simulink model "svpwm_inv_ideal_switch_drive"  (R2025a)
settings: Solver=daessc  StartTime=0.0  StopTime=1  MaxStep=2.5e-7  RelTol=1e-3
model workspace (MAT data in the model file):
  FocDiscrTime = 0.0001
  Is_max = 450
  Ld = 0.00031
  Lq = 0.000305
  PolePairs = 11
  Psi = 0.09569
  Rs = 0.02
  VDC = 400
  compensate_dt = 0
  compensate_pwm = 0
  piBandwidth = 5000
undefined symbols (not defined in the file): Down, Up
libraries: fl_lib x20, nesl_utility x19, ee_lib x15, mcbeeMathTransformLib x7, spsMeanLib x7, slpidlib x5, eePwmGenerator x3, spsRMSLib x2, simulink x2, simulink_extras x1
(part 1 of 2)
settings Model: SimulationMode=rapid-accelerator  ExtModeTrigDuration=100  ParameterArgumentNames=FocDiscrTime  Creator=alexey  LastModifiedBy=alexey
settings SolverCC: ZeroCrossAlgorithm=Adaptive
settings OptimizationCC: DefaultParameterBehavior=Inlined  UseDivisionForNetSlopeComputation=on  GainParamInheritBuiltInType=on  UseFloatMulNetSlope=on  InlineInvariantSignals=on  ReuseModelBlockBuffer=off  EfficientFloat2IntCast=on  LifeSpan=1
settings DebuggingCC: IgnoredZcDiagnostic=none
settings HardwareCC: ProdLongLongMode=on
settings SFSimCC: MATLABDynamicMemAlloc=off
settings RTWCC: GenerateReport=on  LaunchReport=on  GPUComputeCapability=3.5
settings CodeAppCC: ForceParamTrailComments=on
settings GRTTargetCC: RTWCAPISignals=on  RTWCAPIParams=on  CombineSignalStateStructs=on  MatFileLogging=off  SupportVariableSizeSignals=on

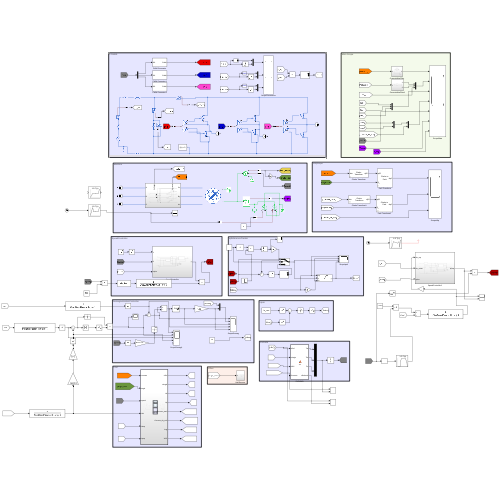
[thumbnail: Simulink's stored preview of the top-level diagram]
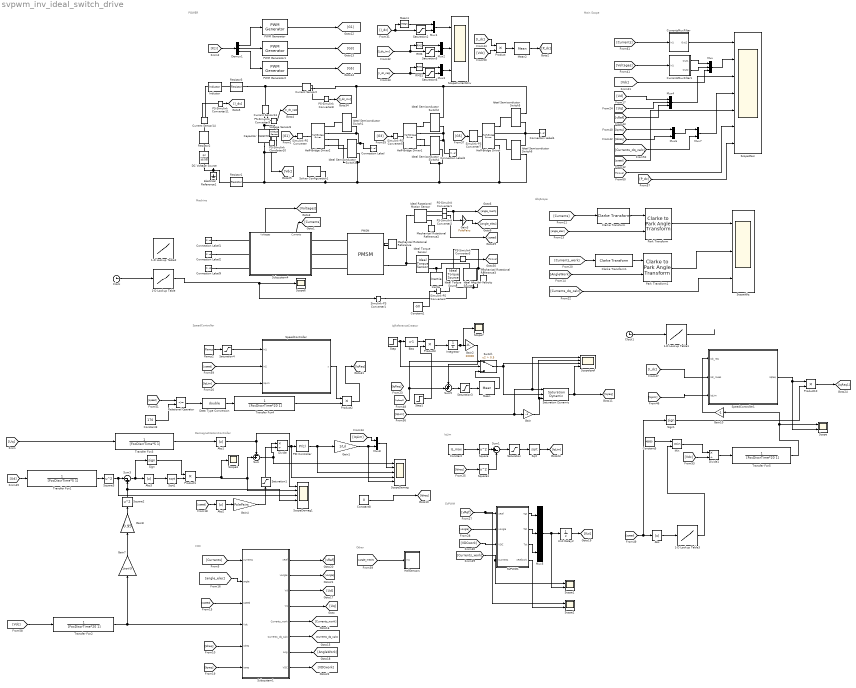
== system svpwm_inv_ideal_switch_drive ==
  note: POWER
  note: IqLim
  note: DemagnetizationController
  note: FOC
  note: Machine
  note: SpeedController
  note: Other
  note: Main Scope
  note: IqReferenceCreator
  note: IdIqScope
  note: SVPWM
  1-D Lookup Table : Lookup_n-D  NumberOfTableDimensions=1  BreakpointsForDimension1=[0 0.4 0.45 0.55 0.87 1 1.5 1.6 1.7]  Table=[0 208 208 104 104 120 120 220 220]  InternalRulePriority=Speed  RndMeth=Simplest
  1-D Lookup Table1 : Lookup_n-D  NumberOfTableDimensions=1  BreakpointsForDimension1=[0 0.3 1 1.2 1.3 1.4 1.5]  Table=[0 200 150 200 30 250 250]  InternalRulePriority=Speed  RndMeth=Simplest
  1-D Lookup Table2 : Lookup_n-D  NumberOfTableDimensions=1  BreakpointsForDimension1=[0 0.4 0.45 0.55 0.87 1 1.5 1.6 1.7]  Table=[0 104 104 104 104 120 120 220 220]  InternalRulePriority=Speed  RndMeth=Simplest
  1-D Lookup Table3 : Lookup_n-D  NumberOfTableDimensions=1  BreakpointsForDimension1=[0 550 600 1000 1925 2350 2400 2450]*0.1047  Table=[0 0 30000 48500 48500 22000 0 0]  InternalRulePriority=Speed  RndMeth=Simplest
  Abs{,1..3} (4 alike) : Abs  SaturateOnIntegerOverflow=off
  Bias : Bias  Bias=-1  SaturateOnIntegerOverflow=off
  Capacitor : fl_lib/Electrical/Electrical Elements/Capacitor  c=300 uF  r=1 mOhm  g=0 1/Ohm  i_specify=off  i_priority=None  i=0 A  i_nominal_specify=off  i_nominal_value=1  i_nominal_unit=A  v_specify=off  v_priority=High  v=400 V  v_nominal_specify=off  v_nominal_value=1  v_nominal_unit=V  vc_specify=on  vc_priority=High  vc=VDC V  vc_nominal_specify=off  vc_nominal_value=1  vc_nominal_unit=V
  Clarke Transform : mcbeeMathTransformLib/Clarke Transform  VariantControl=Variant2  PowerInvariant=off  UseWithEmbedded=on  PhaseInput=Three inputs
      settings: LibrarySourceBlock=mcbcontrolslib/Clarke Transform
  Clarke Transform1 : mcbeeMathTransformLib/Clarke Transform  VariantControl=Variant2  PowerInvariant=off  UseWithEmbedded=on  PhaseInput=Three inputs
      settings: LibrarySourceBlock=mcbcontrolslib/Clarke Transform
  Clock : Clock
  Clock1 : Clock
  Connection Label : ConnectionLabel  Label=A
  Connection Label1 : ConnectionLabel  Label=A
  Connection Label2 : ConnectionLabel  Label=B
  Connection Label3 : ConnectionLabel  Label=B
  Connection Label4 : ConnectionLabel  Label=C
  Connection Label9 : ConnectionLabel  Label=C
  Constant : Constant  Value=Is_max
  Constant1 : Constant  Value=-50
  Constant3 : Constant  Value=170
  Constant5 : Constant  Value=48500
  Constant8 : Constant  Value=0
  Current Sensor13 : fl_lib/Electrical/Electrical Sensors/Current Sensor
  Current Sensor14 : fl_lib/Electrical/Electrical Sensors/Current Sensor
  Current Sensor2 : fl_lib/Electrical/Electrical Sensors/Current Sensor
  CurrentsMuxFilter : Subsystem
  CurrentsMuxFilter1 : Subsystem
  DC Voltage Source : ee_lib/Additional Components/SPICE Sources/DC Voltage Source  DC=VDC V
  Data Type Conversion : DataTypeConversion  OutDataTypeStr=double  SaturateOnIntegerOverflow=off  RndMeth=Floor
  Demux1 : Demux  Outputs=3
  Divide : Product  Inputs=*/
  Divide1 : Product  Inputs=*/
  Electrical Reference1 : fl_lib/Electrical/Electrical Elements/Electrical Reference
  Gain : Gain  Gain=-1
  Gain1 : Gain  Gain=1/Ld
  Gain10 : Gain  Gain=-1
  Gain2 : Gain  Gain=20000
  Gain3 : Gain  Gain=PolePairs
  Gain4 : Gain  Gain=PolePairs
  Gain7 : Gain  Gain=1/sqrt(3)
  Gain8 : Gain  Gain=0.95
  Half-Bridge Driver : ee_lib/Semiconductors & Converters/Half-Bridge Driver  port_option=ee.enum.controlport.ps  uHigh=2.0 V  uLow=0.8 V  uHighValue=0.7  uLowValue=0.3  vHigh=15 V  vLow=0 V  tpLH=50 ns  tdLH=1 ns  tpHL=50 ns  tdHL=1 ns  parameterization=ee.enum.semiconductors.gateDriverParam.outputImpedance  rHigh=2 Ohm  rLow=2 Ohm  tRise=20 ns  tFall=20 ns  cLoad=10 nF  ZonTime_specify=off  ZonTime_priority=None  ZonTime=0 s  ZoffTime_specify=off  ZoffTime_priority=None  ZoffTime=0 s  power_dissipated_high_side_specify=off  power_dissipated_high_side_priority=None  power_dissipated_high_side=0 W  power_dissipated_high_side_nominal_specify=off  power_dissipated_high_side_nominal_value=1  power_dissipated_high_side_nominal_unit=W  power_dissipated_low_side_specify=off  power_dissipated_low_side_priority=None  power_dissipated_low_side=0 W  power_dissipated_low_side_nominal_specify=off  power_dissipated_low_side_nominal_value=1  power_dissipated_low_side_nominal_unit=W
      settings: InternalSimscapePortConfiguration="{\"Bottom\":[],\"Left\":[{\"id\":\"u\",\"label\":\"u\",\"type\":\"input\"}],\"Right\":[{\"id\":\"HO\",\"label\":\"HO\",\"type\":\"foundation.electrical.electrical\"},{\"id\":\"HS\",\"label\":\"HS\",\"type\":\"foundation.electrical.electrical\"},{\"id\":\"LO\",\"label\":\"LO\",\"type\":\"foundation.electrical.electrical\"},{\"id\":\"LS\",\"label\":\"LS\",\"type\":\"foundation.electrical.electrical\"}],\"Top\":[]}"
  Half-Bridge Driver1 : ee_lib/Semiconductors & Converters/Half-Bridge Driver  port_option=ee.enum.controlport.ps  uHigh=2.0 V  uLow=0.8 V  uHighValue=0.7  uLowValue=0.3  vHigh=15 V  vLow=0 V  tpLH=50 ns  tdLH=1 ns  tpHL=50 ns  tdHL=1 ns  parameterization=ee.enum.semiconductors.gateDriverParam.outputImpedance  rHigh=2 Ohm  rLow=2 Ohm  tRise=20 ns  tFall=20 ns  cLoad=10 nF  ZonTime_specify=off  ZonTime_priority=None  ZonTime=0 s  ZoffTime_specify=off  ZoffTime_priority=None  ZoffTime=0 s  power_dissipated_high_side_specify=off  power_dissipated_high_side_priority=None  power_dissipated_high_side=0 W  power_dissipated_high_side_nominal_specify=off  power_dissipated_high_side_nominal_value=1  power_dissipated_high_side_nominal_unit=W  power_dissipated_low_side_specify=off  power_dissipated_low_side_priority=None  power_dissipated_low_side=0 W  power_dissipated_low_side_nominal_specify=off  power_dissipated_low_side_nominal_value=1  power_dissipated_low_side_nominal_unit=W
      settings: InternalSimscapePortConfiguration="{\"Bottom\":[],\"Left\":[{\"id\":\"u\",\"label\":\"u\",\"type\":\"input\"}],\"Right\":[{\"id\":\"HO\",\"label\":\"HO\",\"type\":\"foundation.electrical.electrical\"},{\"id\":\"HS\",\"label\":\"HS\",\"type\":\"foundation.electrical.electrical\"},{\"id\":\"LO\",\"label\":\"LO\",\"type\":\"foundation.electrical.electrical\"},{\"id\":\"LS\",\"label\":\"LS\",\"type\":\"foundation.electrical.electrical\"}],\"Top\":[]}"
  Half-Bridge Driver2 : ee_lib/Semiconductors & Converters/Half-Bridge Driver  port_option=ee.enum.controlport.ps  uHigh=2.0 V  uLow=0.8 V  uHighValue=0.7  uLowValue=0.3  vHigh=15 V  vLow=0 V  tpLH=50 ns  tdLH=1 ns  tpHL=50 ns  tdHL=1 ns  parameterization=ee.enum.semiconductors.gateDriverParam.outputImpedance  rHigh=2 Ohm  rLow=2 Ohm  tRise=20 ns  tFall=20 ns  cLoad=10 nF  ZonTime_specify=off  ZonTime_priority=None  ZonTime=0 s  ZoffTime_specify=off  ZoffTime_priority=None  ZoffTime=0 s  power_dissipated_high_side_specify=off  power_dissipated_high_side_priority=None  power_dissipated_high_side=0 W  power_dissipated_high_side_nominal_specify=off  power_dissipated_high_side_nominal_value=1  power_dissipated_high_side_nominal_unit=W  power_dissipated_low_side_specify=off  power_dissipated_low_side_priority=None  power_dissipated_low_side=0 W  power_dissipated_low_side_nominal_specify=off  power_dissipated_low_side_nominal_value=1  power_dissipated_low_side_nominal_unit=W
      settings: InternalSimscapePortConfiguration="{\"Bottom\":[],\"Left\":[{\"id\":\"u\",\"label\":\"u\",\"type\":\"input\"}],\"Right\":[{\"id\":\"HO\",\"label\":\"HO\",\"type\":\"foundation.electrical.electrical\"},{\"id\":\"HS\",\"label\":\"HS\",\"type\":\"foundation.electrical.electrical\"},{\"id\":\"LO\",\"label\":\"LO\",\"type\":\"foundation.electrical.electrical\"},{\"id\":\"LS\",\"label\":\"LS\",\"type\":\"foundation.electrical.electrical\"}],\"Top\":[]}"
  HallSensors : Subsystem
  Ideal Angular Velocity Source : fl_lib/Mechanical/Mechanical Sources/Ideal Angular Velocity Source
  Ideal Rotational Motion Sensor : fl_lib/Mechanical/Mechanical Sensors/Ideal Rotational Motion Sensor  reference=foundation.enum.MeasurementReference.difference  acceleration_port=false  velocity_port=true  position_port=true  wrap_angle=false  offset=0 rad
  Ideal Semiconductor Switch{1..6} (6 alike) : ee_lib/Semiconductors & Converters/Ideal Semiconductor Switch  port_option=ee.enum.controlport.elec  Ron=0.0001 Ohm  Goff=1e-6 1/Ohm  Vth=10 V  diode_param=ee.enum.semiconductors.protectionDiode.nodynamics  diode_Vf=0.8 V  diode_Ron=0.001 Ohm  diode_Goff=1e-5 1/Ohm  diode_C=50e-9 F  diode_iRM=-235 A  diode_iF=300 A  diode_idot=-50 A/us  diode_trr_param=ee.enum.converters.diodetrr.trr_factor  diode_trr_factor=3  diode_trr=15 us  diode_Qrr=1500 s*uA
      settings: InternalSimscapePortConfiguration="{\"Bottom\":[],\"Left\":[{\"id\":\"G_elec\",\"label\":\"\",\"type\":\"foundation.electrical.electrical\"}],\"Right\":[{\"id\":\"A\",\"label\":\"a\",\"type\":\"foundation.electrical.electrical\"},{\"id\":\"K\",\"label\":\"k\",\"type\":\"foundation.electrical.electrical\"}],\"Top\":[]}"
  Ideal Torque Sensor : fl_lib/Mechanical/Mechanical Sensors/Ideal Torque Sensor
  Ideal Torque Source : fl_lib/Mechanical/Mechanical Sources/Ideal Torque Source
  Inductor : ee_lib/Passive/Inductor  l=220e-9 H  enable_L_tol=ee.enum.toleranceApplication.none  L_tol=20  tol_distribution=ee.enum.toleranceDistribution.uniform  nSigma=4  r=0 Ohm  g=1e-9 1/Ohm  enable_operating_limits=ee.enum.enable.no  operating_limit_action=ee.enum.passive.reportOpLim.warn  max_working_current=1 A  power_rating=1 W  i_L_specify=off  i_L_priority=High  i_L=0 A  i_L_nominal_specify=off  i_L_nominal_value=1  i_L_nominal_unit=A
  Inertia : fl_lib/Mechanical/Rotational Elements/Inertia  inertia=0.1 kg*m^2  num_ports=foundation.enum.numPorts2.one  w_specify=off  w_priority=High  w=0 rad/s  w_nominal_specify=off  w_nominal_value=1  w_nominal_unit=rad/s  t_specify=off  t_priority=None  t=0 N*m  t_nominal_specify=off  t_nominal_value=1  t_nominal_unit=N*m
  Integrator : Integrator  LimitOutput=on  UpperSaturationLimit=0  LowerSaturationLimit=-2*Is_max/20000
  Mean : spsMeanLib/Mean  Freq=1000  Vinit=0  Ts=0
  Mean1 : spsMeanLib/Mean  Freq=1/FocDiscrTime/20  Vinit=0  Ts=0
  Mean2 : spsMeanLib/Mean  Freq=1/FocDiscrTime/20  Vinit=0  Ts=0
  Mechanical Rotational Reference : fl_lib/Mechanical/Rotational Elements/Mechanical Rotational Reference
  Mechanical Rotational Reference2 : fl_lib/Mechanical/Rotational Elements/Mechanical Rotational Reference
  Mechanical Rotational Reference3 : fl_lib/Mechanical/Rotational Elements/Mechanical Rotational Reference
  Min : MinMax  Inputs=2
  Mux : Mux  Inputs=3
  Mux{1..3,6..8} (6 alike) : Mux  Inputs=2
  Mux4 : Mux  Inputs=3
  Mux5 : Mux  Inputs=3
  PID Controller : slpidlib/PID Controller  Controller=PI  Form=Parallel  TimeDomain=Discrete-time  UseExternalTs=off  SampleTime=FocDiscrTime*10  IntegratorMethod=Forward Euler  FilterMethod=Forward Euler  ControllerParametersSource=internal  P=0.1*5  I=100*5  UseKiTs=off  D=0.01  UseExternalDerivativeSource=off  N=100  UseFilter=on  TunerSelectOption=Transfer Function Based (PID Tuner App)  InitialConditionSource=internal  InitialConditionForIntegrator=0  InitialConditionForFilter=0  DifferentiatorICPrevScaledInput=0  ExternalReset=none  TrackingMode=off  Kt=1  LimitOutput=on  SatLimitsSource=internal  UpperSaturationLimit=0  LowerSaturationLimit=-300*Ld  LinearizeAsGain=on  AntiWindupMode=clamping  Kb=1  LimitIntegrator=off  UpperIntegratorSaturationLimit=inf  LowerIntegratorSaturationLimit=-inf  POutMin=[]  POutMax=[]  IOutMin=[]  IOutMax=[]  DOutMin=[]  DOutMax=[]  NOutMin=[]  NOutMax=[]  SumOutMin=[]  SumOutMax=[]  SaturationOutMin=[]  SaturationOutMax=[]  PParamMin=[]  PParamMax=[]  IParamMin=[]  IParamMax=[]  DParamMin=[]  DParamMax=[]  NParamMin=[]  NParamMax=[]  KbParamMin=[]  KbParamMax=[]  KtParamMin=[]  KtParamMax=[]  KbOutMin=[]  KbOutMax=[]  KtOutMin=[]  KtOutMax=[]  IntegratorOutMin=[]  IntegratorOutMax=[]  FilterOutMin=[]  FilterOutMax=[]  SumI1OutMin=[]  SumI1OutMax=[]  SumI2OutMin=[]  SumI2OutMax=[]  SumI3OutMin=[]  SumI3OutMax=[]  SumI4OutMin=[]  SumI4OutMax=[]  SumDOutMin=[]  SumDOutMax=[]  DifferentiatorOutMin=[]  DifferentiatorOutMax=[]  FilterDiffOutCoefMin=[]  FilterDiffOutCoefMax=[]  ReciprocalOutMin=[]  ReciprocalOutMax=[]  SumDenOutMin=[]  SumDenOutMax=[]  SumNumOutMin=[]  SumNumOutMax=[]  DivideOutMin=[]  DivideOutMax=[]  UdiffTsProdOutMin=[]  UdiffTsProdOutMax=[]  NTsProdOutMin=[]  NTsProdOutMax=[]  UintegralTsProdOutMin=[]  UintegralTsProdOutMax=[]  UngainTsProdOutMin=[]  UngainTsProdOutMax=[]  ClampingZeroOutDataTypeStr=Inherit: Inherit via back propagation  ClampingZeroOutMin=[]  ClampingZeroOutMax=[]  FilterDenConstantOutDataTypeStr=Inherit: Inherit via back propagation  FilterDenConstantOutMin=[]  FilterDenConstantOutMax=[]  PCopyOutDataTypeStr=Inherit: Inherit via back propagation  PCopyOutMin=[]  PCopyOutMax=[]  NCopyOutDataTypeStr=Inherit: Inherit via back propagation  NCopyOutMin=[]  NCopyOutMax=[]  IntegratorContinuousStateAttributes=''  IntegratorStateMustResolveToSignalObject=off  IntegratorRTWStateStorageClass=Auto  FilterContinuousStateAttributes=''  FilterStateMustResolveToSignalObject=off  FilterRTWStateStorageClass=Auto  ParallelPVariant=InternalParameters  IdealPVariant=Disabled  IVariant=InternalParameters  DVariant=Disabled  IntegratorVariant=Discrete  SatVariant=Enabled  AWVariant=DiscClampingParallel  PCopyVariant=Disabled  TRVariant=Disabled  FdbkBlocksVariant=Forward  IdealPFdbkVariant=Disabled  SatFdbkVariant=Disabled  DerivativeFilterVariant=Disabled  NVariant=Disabled  NCopyVariant=Disabled_SignalSpec  FilterICVariant=Disabled  IntegratorICVariant=InternalICs  ExternalResetVariant=Disabled  TRSumVariant=Passthrough  SumFdbkVariant=Disabled  SumVariant=Sum_PI  TsampFilterVariant=InternalTs  TsampNgainVariant=Passthrough  TsampIntegralVariant=Disabled_SignalSpec  ExternalSaturationOutDataTypeStr=Inherit: Same as second input  DerivativeSourceVariant=Disabled  PreIntVariant=InternalPreInt
  PMSM : ee_lib/Electromechanical/Permanent Magnet/PMSM  port_option=ee.enum.threePhasePort.expanded  winding_type=ee.enum.electromech.statorconfiguration.wye  machine_param=ee.enum.pmsm.parameterization.constant  nPolePairs=PolePairs  pmflux_param=ee.enum.pmflux.fluxlinkage  pm_flux_linkage=Psi Wb  torque_constant=0.074 N*m/A  back_emf_constant=0.06 V*s/rad  stator_param=ee.enum.statorparam.LdLqL0  Ld=Ld H  Lq=Lq H  idVec=[-200, 0, 200] A  iqVec=[-200, 0, 200] A  LdMatrix=0.0002 * ones(3, 3) H  LqMatrix=0.0002 * ones(3, 3) H  PmMatrix=0.1 * ones(3, 3) Wb  ktMatrix=0.18 * ones(3, 3) N*m/A  keMatrix=0.18 * ones(3, 3) V*s/rad  L0=1e-6 uH  Ls=0.0002 H  Lm=-0.00002 H  Ms=0.00002 H  Rs=Rs Ohm  zero_sequence=ee.enum.park.zerosequence.exclude  axes_param=ee.enum.rotorangle.daxis  loss_param=ee.enum.ironloss.none  losses_oc=[0, 0, 0] W  losses_sc=[0, 0, 0] W  f_losses=60 Hz  Isc_losses=95 A  J=0 kg*m^2  lam=0 N*m*s/rad  i_d_specify=on  i_d_priority=High  i_d=0 A  i_d_nominal_specify=off  i_d_nominal_value=1  i_d_nominal_unit=A  i_q_specify=on  i_q_priority=High  i_q=0 A  i_q_nominal_specify=off  i_q_nominal_value=1  i_q_nominal_unit=A  torque_specify=on  torque_priority=High  torque=0 N*m  torque_nominal_specify=off  torque_nominal_value=1  torque_nominal_unit=N*m  angular_velocity_specify=on  angular_velocity_priority=None  angular_velocity=7000 rpm  angular_velocity_nominal_specify=off  angular_velocity_nominal_value=1  angular_velocity_nominal_unit=rpm  angular_position_specify=on  angular_position_priority=High  angular_position=0 deg  angular_position_nominal_specify=off  angular_position_nominal_value=1  angular_position_nominal_unit=deg  alpha=3.93e-3 1/K  alpha_flux=-0.001 1/K  Tmeas=298.15 K  stator_thermal_mass=100 J/K  rotor_thermal_mass=200 J/K  Rm_percent_rotor=90  Rd_percent_rotor=30  temperatureA_specify=off  temperatureA_priority=High  temperatureA=25 degC  temperatureA_nominal_specify=off  temperatureA_nominal_value=1  temperatureA_nominal_unit=degC  temperatureB_specify=off  temperatureB_priority=High  temperatureB=25 degC  temperatureB_nominal_specify=off  temperatureB_nominal_value=1  temperatureB_nominal_unit=degC  temperatureC_specify=off  temperatureC_priority=High  temperatureC=25 degC  temperatureC_nominal_specify=off  temperatureC_nominal_value=1  temperatureC_nominal_unit=degC  temperatureR_specify=off  temperatureR_priority=High  temperatureR=25 degC  temperatureR_nominal_specify=off  temperatureR_nominal_value=1  temperatureR_nominal_unit=degC
      settings: InternalSimscapePortConfiguration="{\"Bottom\":[],\"Left\":[{\"id\":\"a\",\"label\":\"a\",\"type\":\"foundation.electrical.electrical\"},{\"id\":\"b\",\"label\":\"b\",\"type\":\"foundation.electrical.electrical\"},{\"id\":\"c\",\"label\":\"c\",\"type\":\"foundation.electrical.electrical\"}],\"Right\":[{\"id\":\"R\",\"label\":\"R\",\"type\":\"foundation.mechanical.rotational.rotational\"},{\"id\":\"C\",\"label\":\"C\",\"type\":\"foundation.mechanical.rotational.rotational\"}],\"Top\":[]}"
  PS-Simulink Converter{1..3,8..11} (7 alike) : nesl_utility/PS-Simulink Converter  PhysicalDomain=network_engine_domain  SubClassName=ps_output  LeftPortType=input  RightPortType=output  PseudoPeriodic=off  Frequencies=[]  VectorFormat=inherit  Unit=inherit  AffineConversion=off
  PWM Generator : eePwmGenerator/PWM Generator  CarrCount=Up-Down  Tper=0.5*FocDiscrTime  Tdelay=FocDiscrTime/2  Ts=50e-9
  PWM Generator1 : eePwmGenerator/PWM Generator  CarrCount=Up-Down  Tper=0.5*FocDiscrTime  Tdelay=FocDiscrTime/2  Ts=50e-9
  PWM Generator2 : eePwmGenerator/PWM Generator  CarrCount=Up-Down  Tper=0.5*FocDiscrTime  Tdelay=FocDiscrTime/2  Ts=50e-9
  Park Transform : mcbeeMathTransformLib/Clarke to Park Angle Transform  AxisAlignment=D-axis  UseWithEmbedded=on  PhaseInput=Three inputs  ThetaInput=Electrical position  AngleInput=Radians  N_points=1024
      settings: LibrarySourceBlock=mcbcontrolslib/Park Transform
  Park Transform1 : mcbeeMathTransformLib/Clarke to Park Angle Transform  AxisAlignment=D-axis  UseWithEmbedded=on  PhaseInput=Three inputs  ThetaInput=Electrical position  AngleInput=Radians  N_points=1024
      settings: LibrarySourceBlock=mcbcontrolslib/Park Transform
  Product{,1..3,10} (5 alike) : Product
  RMS : spsRMSLib/RMS  TrueRMS=on  Freq=1/FocDiscrTime/20  RMSInit=0  Ts=0
  RMS1 : spsRMSLib/RMS  TrueRMS=on  Freq=1/FocDiscrTime/20  RMSInit=0  Ts=0
  Ramp2 : simulink/Sources/Ramp  slope=300/4e-3  start=1e-3  InitialOutput=0
  Relational Operator : RelationalOperator  Operator=<=  OutDataTypeStr=boolean  RndMeth=Simplest  InputSameDT=off
  Resistor1 : ee_lib/Passive/Resistor  R=1 mOhm  enable_R_tol=0  R_tol=5  tol_distribution=1  nSigma=4  enable_operating_limits=0  operating_limit_action=2  power_rating=1 W  max_working_voltage=100 V  noise_mode=0  Tdevice=25 degC  sample_time=1e-3 s  repeatability=1  user_seed=0  auto_seed=3890346746  power_derating_T1=70 degC  power_derating_T2=155 degC  operating_temperature_range_vec=[-50, 150] degC  alpha=3.93e-3 1/K  Tmeas=25 degC  thermal_mass=100 J/K  temperature_specify=off  temperature_priority=High  temperature=298.15 K  temperature_nominal_specify=off  temperature_nominal_value=1  temperature_nominal_unit=K
  Resistor2 : ee_lib/Passive/Resistor  R=70 mOhm  enable_R_tol=0  R_tol=5  tol_distribution=1  nSigma=4  enable_operating_limits=0  operating_limit_action=2  power_rating=1 W  max_working_voltage=100 V  noise_mode=0  Tdevice=25 degC  sample_time=1e-3 s  repeatability=1  user_seed=0  auto_seed=3474941853  power_derating_T1=70 degC  power_derating_T2=155 degC  operating_temperature_range_vec=[-50, 150] degC  alpha=3.93e-3 1/K  Tmeas=25 degC  thermal_mass=100 J/K  temperature_specify=off  temperature_priority=High  temperature=298.15 K  temperature_nominal_specify=off  temperature_nominal_value=1  temperature_nominal_unit=K
  Resistor3 : ee_lib/Passive/Resistor  R=5 mOhm  enable_R_tol=0  R_tol=5  tol_distribution=1  nSigma=4  enable_operating_limits=0  operating_limit_action=2  power_rating=1 W  max_working_voltage=100 V  noise_mode=0  Tdevice=25 degC  sample_time=1e-3 s  repeatability=1  user_seed=0  auto_seed=545404223  power_derating_T1=70 degC  power_derating_T2=155 degC  operating_temperature_range_vec=[-50, 150] degC  alpha=3.93e-3 1/K  Tmeas=25 degC  thermal_mass=100 J/K  temperature_specify=off  temperature_priority=High  temperature=298.15 K  temperature_nominal_specify=off  temperature_nominal_value=1  temperature_nominal_unit=K
  SVPWM1 : MATLAB Function  TreatAsAtomicUnit=on  SystemSampleTime=FocDiscrTime/2
  Saturation : Saturate  UpperLimit=inf  LowerLimit=0
  Saturation Dynamic : simulink/Discontinuities/Saturation Dynamic  OutMin=[]  OutMax=[]  OutDataTypeStr=Inherit: Same as second input  OutDataType=fixdt(1, 16)  OutScaling=2^-10  DoSatur=off
  Saturation1 : Saturate  UpperLimit=inf  LowerLimit=1
  Saturation2 : Saturate  UpperLimit=500  LowerLimit=-500
  Saturation3 : Saturate  UpperLimit=inf  LowerLimit=-Is_max
  Saturation4 : Saturate  UpperLimit=600  LowerLimit=0
  Saturation5 : Saturate  UpperLimit=500  LowerLimit=-500
  Saturation6 : Saturate  UpperLimit=500  LowerLimit=-500
  Scope : Scope  NumInputPorts=2
      settings: ActiveDisplayYMinimum=-15.059619746885231  ActiveDisplayYMaximum=135.53657772196712  DataLoggingVariableName=ScopeData18
  Scope1 : Scope  NumInputPorts=2
      settings: ActiveDisplayYMinimum=-438.55416313604536  ActiveDisplayYMaximum=438.95198817062709  DataLoggingVariableName=ScopeData14
  Scope2 : Scope  NumInputPorts=2
      settings: ActiveDisplayYMinimum=192.19580526011231  ActiveDisplayYMaximum=251.38218785320146  DataLoggingVariableName=ScopeData2
  Scope3 : Scope
      settings: ActiveDisplayYMinimum=-26.205212969517383  ActiveDisplayYMaximum=235.84691672565651  DataLoggingVariableName=ScopeData12
  Scope6 : Scope
      settings: ActiveDisplayYMinimum=-68.247393749999986  ActiveDisplayYMaximum=614.22654375  DataLoggingVariableName=ScopeData15
  Scope7 : Scope
      settings: DataLoggingVariableName=ScopeData16
  ScopeCurrentsInv : Scope  NumInputPorts=3
      settings: ActiveDisplayString=3  ActiveDisplayYMinimum=-395.16223848004176  ActiveDisplayYMaximum=599.4624709422269  DataLoggingVariableName=ScopeData8
  ScopeDemag : Scope  NumInputPorts=5
      settings: ActiveDisplayYMinimum=-32.502064809215938  ActiveDisplayYMaximum=292.5185832829435  DataLoggingVariableName=ScopeData7
  ScopeDemag1 : Scope  NumInputPorts=5
      settings: ActiveDisplayYMinimum=-1.4930057665002543  ActiveDisplayYMaximum=13.43705189850229  DataLoggingVariableName=ScopeData17
  ScopeIdIq : Scope  NumInputPorts=3
      settings: ActiveDisplayYMinimum=-106.63997343508196  ActiveDisplayYMaximum=61.771427764004578  DataLoggingVariableName=ScopeData13
  ScopeIqref : Scope  NumInputPorts=4
      settings: ActiveDisplayYMinimum=350  ActiveDisplayYMaximum=550  DataLoggingVariableName=ScopeData11
  ScopeMain : Scope  NumInputPorts=7
      settings: ActiveDisplayString=4  ActiveDisplayYMinimum=-544.57327394438  ActiveDisplayYMaximum=401.15946549942004  DataLoggingVariableName=ScopeData9
  Sign : Signum
  Sign1 : Signum
  Simulink-PS Converter : nesl_utility/Simulink-PS Converter  PhysicalDomain=network_engine_domain  SubClassName=ps_input  LeftPortType=input  RightPortType=output  PseudoPeriodic=off  Frequencies=[]  NoiseDistribution=none  NoiseParameters=[]  Unit=1  AffineConversion=off  FilteringAndDerivatives=provide  SimscapeFilterOrder=1  InputFilterTimeConstant=0.001  UdotUserProvided=0
  Simulink-PS Converter1 : nesl_utility/Simulink-PS Converter  PhysicalDomain=network_engine_domain  SubClassName=ps_input  LeftPortType=input  RightPortType=output  PseudoPeriodic=off  Frequencies=[]  NoiseDistribution=none  NoiseParameters=[]  Unit=1  AffineConversion=off  FilteringAndDerivatives=filter  SimscapeFilterOrder=1  InputFilterTimeConstant=1e-3  UdotUserProvided=0
  Simulink-PS Converter2 : nesl_utility/Simulink-PS Converter  PhysicalDomain=network_engine_domain  SubClassName=ps_input  LeftPortType=input  RightPortType=output  PseudoPeriodic=off  Frequencies=[]  NoiseDistribution=none  NoiseParameters=[]  Unit=1  AffineConversion=off  FilteringAndDerivatives=filter  SimscapeFilterOrder=1  InputFilterTimeConstant=1e-3  UdotUserProvided=0
  Simulink-PS Converter5 : nesl_utility/Simulink-PS Converter  PhysicalDomain=network_engine_domain  SubClassName=ps_input  LeftPortType=input  RightPortType=output  PseudoPeriodic=off  Frequencies=[]  NoiseDistribution=none  NoiseParameters=[]  Unit=1  AffineConversion=off  FilteringAndDerivatives=provide  SimscapeFilterOrder=1  InputFilterTimeConstant=0.001  UdotUserProvided=0
  Simulink-PS Converter7 : nesl_utility/Simulink-PS Converter  PhysicalDomain=network_engine_domain  SubClassName=ps_input  LeftPortType=input  RightPortType=output  PseudoPeriodic=off  Frequencies=[]  NoiseDistribution=none  NoiseParameters=[]  Unit=1  AffineConversion=off  FilteringAndDerivatives=provide  SimscapeFilterOrder=1  InputFilterTimeConstant=0.001  UdotUserProvided=0
  Solver Configuration1 : nesl_utility/Solver Configuration  PhysicalDomain=network_engine_domain  SubClassName=solver  LeftPortType=input  RightPortType=generic  Tones=[]  Harmonics=[]  SimulateNoise=off  Profile=off  UseLocalSampling=off  EnableSwitchedLinearOptims=on  FrequencyDomain=off  UseCCode=off  RelTol=0.001  AbsTol=0.001  MinStep=1e-09  ToWorkspace=off  RevertToSquareIcSolve=off  NumHomotopyIterations=100  PhasorMode=off  PhasorModeNumHarmonics=1  ConsistencySolver=NEWTON_XTOL_AFTER_FTOL  IndexReductionMethod=DerivativeReplacement  DoDC=off  ResidualTolerance=1e-09  ConsistencyTolSource=GLOBAL  ConsistencyAbsTol=0.001  ConsistencyRelTol=0.001  ConsistencyTolFactor=0.001  UseLocalSolver=off  LocalSolverChoice=NE_BACKWARD_EULER_ADVANCER  ResolveIndetEquations=on  FunctionEvalNumThread=1  LocalSolverSampleTime=0.001  DoFixedCost=off  MaxNonlinIter=3  MaxModeIter=2  ComputeImpulses=off  ImpulseIterations=2  LinearAlgebra=auto  LinearAlgebraNumThread=0  EquationFormulation=NE_TIME_EF  DelaysMemoryBudget=1024  AutomaticFiltering=on  FilteringTimeConstant=0.001  PartitionStorageMethod=AS_NEEDED  PartitionMemoryBudget=1024  PartitionMethod=ROBUST  MultibodyUseLocalSolver=off  MultibodyLocalSolverChoice=ODE1  MultibodyLocalSolverSampleTime=0.001
  SpeedController : Subsystem
  SpeedController1 : Subsystem
  Sqrt : Sqrt
  Sqrt1 : Sqrt
  Square{,1..3} (4 alike) : Math  Operator=square
  Step : Step  Time=2  Before=1  After=0  SampleTime=0
  Step1 : Step  Time=0.7  Before=1  After=-1  SampleTime=0
  Subsystem1 : Subsystem  TreatAsAtomicUnit=on  SystemSampleTime=FocDiscrTime
  Subsystem4 : Subsystem
      settings: PortSchema="{\"entries\":[{\"content\":{\"sides\":[{\"content\":{},\"type\":\"ConnectorPlacement.EquallySpacedRectSide\",\"uuid\":\"18ff9a98-da5f-4d42-bf88-8b80acaefaab\"},{\"content\":{\"connectorIds\":[\"Out1\",\"Out2\"],\"side\":\"RIGHT\"},\"type\":\"ConnectorPlacement.EquallySpacedRectSide\",\"uuid\":\"2ae2e449-c022-4e43-8d74-e7903f555369\"},{\"content\":{\"connectorIds\":[\"LConn1\",\"LConn2\",\"LConn3\"],\"side\":\"TOP\"},\"type\":\"ConnectorPlacement.EquallySpacedRectSide\",\"uuid\":\"55b123c9-903d-428f-ba92-02a5913ccae5\"},{\"content\":{\"connectorIds\":[\"RConn1\",\"RConn2\",\"RConn3\"],\"side\":\"BOTTOM\"},\"type\":\"ConnectorPlacement.EquallySpacedRectSide\",\"uuid\":\"b028b0af-4fd3-4535-8d3b-f50dc0cabb29\"}]},\"type\":\"ConnectorPlacement.EquallySpacedConnector\",\"uuid\":\"08d0fd08-360e-4301-974e-a78b2c2bf0b9\"}],\"packageUris\":[\"http://schema.mathworks.com/mf0/Connector/R2020b\"],\"version\":\"1.0\"}"
  Sum : Sum  Inputs=-+|
  Sum1 : Sum  Inputs=|+-
  Sum3 : Sum  Inputs=|-+
  Sum5 : Sum  Inputs=++|
  Switch : Switch  Criteria=u2 > Threshold  Threshold=0.5  SaturateOnIntegerOverflow=off  InputSameDT=off
  Transfer Fcn1 : TransferFcn  Denominator=[FocDiscrTime*5 1]
  Transfer Fcn2 : TransferFcn  Denominator=[FocDiscrTime*20 1]
  Transfer Fcn3 : TransferFcn  Denominator=[FocDiscrTime*5 1]
  Transfer Fcn4 : TransferFcn  Denominator=[FocDiscrTime*20 1]
  Transfer Fcn5 : TransferFcn  Denominator=[FocDiscrTime*20 1]
  Unit Delay2 : UnitDelay  SampleTime=FocDiscrTime/2  HasFrameUpgradeWarning=on
  Voltage Sensor8 : fl_lib/Electrical/Electrical Sensors/Voltage Sensor
  wires:
  PS-Simulink Converter9/1 -> [I_dc_cap]
  PS-Simulink Converter10/1 -> [Vdc]
  [G1] -> Simulink-PS Converter/1
  [G5] -> Simulink-PS Converter7/1
  PS-Simulink Converter11/1 -> [I_dc]
  [G3] -> Simulink-PS Converter5/1
  PS-Simulink Converter8/1 -> [I_dc_inv]
  [Kzi] -> Demux1/1
  Demux1/1 -> PWM Generator/1
  Demux1/2 -> PWM Generator1/1
  Demux1/3 -> PWM Generator2/1
  PWM Generator/1 -> [G1]
  PWM Generator1/1 -> [G3]
  PWM Generator2/1 -> [G5]
  [I_dc_inv] -> RMS/1, Saturation5/1
  [I_dc] -> Mean1/1, Saturation2/1
  [I_dc_cap] -> RMS1/1, Saturation6/1
  Mean1/1 -> Mux1/1
  RMS/1 -> Mux2/1
  Mux2/1 -> ScopeCurrentsInv/2
  Mux1/1 -> ScopeCurrentsInv/1
  Mux3/1 -> ScopeCurrentsInv/3
  RMS1/1 -> Mux3/1
  Saturation2/1 -> Mux1/2
  Saturation5/1 -> Mux2/2
  Saturation6/1 -> Mux3/2
  Product2/1 -> [IqReq]
  Clarke Transform1/1 -> Park Transform1/1
  Sum/1 -> Divide/1, ScopeDemag/1
  Sum3/1 -> Abs3/1, Sign/1
  Constant3/1 -> Relational Operator/2
  Product3/1 -> Integrator/1
  Sqrt/1 -> [IqLim]
  [I_dc] -> SpeedController1/2(Idc_meas)
  [Idreq] -> Subsystem1/5(Idreq)
  Abs2/1 -> Gain4/1
  Product/1 -> Mean2/1
  Clock/1 -> 1-D Lookup Table/1
  [VDCwork] -> SVPWM1/3(VDC)
  Constant1/1 -> Simulink-PS Converter2/1
  [angle_mech] -> HallSensors/1(In1)
  PS-Simulink Converter1/1 -> Gain3/1, [angle_mech]
  Park Transform/1 -> ScopeIdIq/1
  1-D Lookup Table/1 -> Simulink-PS Converter1/1, Scope6/1
  SpeedController/1(y) -> Product2/1
  Step1/1 -> Product3/2
  Clarke Transform/1 -> Park Transform/1
  Divide1/1 -> Transfer Fcn5/1
  CurrentsMuxFilter1/2(Out2) -> Mux/2
  CurrentsMuxFilter/1(Out2) -> ScopeMain/1
  Square2/1 -> Sum3/2, ScopeDemag1/4
  SVPWM1/1(Tat) -> Mux5/1
  Abs1/1 -> Sum/1, ScopeDemag1/1
  PID Controller/1 -> ScopeDemag/3, Gain1/1
  Gain7/1 -> Gain8/1
  Gain1/1 -> ScopeDemag/5, Mux8/2
  Product1/1 -> Scope3/1, Sum/2, ScopeDemag1/2
  [Currents] -> Subsystem1/1(currents)
  Gain2/1 -> Sum5/1
  [Vdc] -> Mux/3
  Square3/1 -> ScopeDemag1/3, Sum3/1
  Subsystem1/6(Currents_dq_calc) -> [Currents_dq_calc]
  SVPWM1/2(Tbt) -> Mux5/2
  Saturation Dynamic/1 -> ScopeIqref/4, [Iqreq]
  Subsystem1/4(Vq) -> [Uq]
  Mux6/1 -> Mux7/1
  [Uq] -> Mux4/2
  1-D Lookup Table3/1 -> Min/2
  Divide/1 -> PID Controller/1, ScopeDemag/4
  [Currents_work] -> Clarke Transform1/1
  Product10/1 -> [IqReq1]
  [speed] -> Abs2/1
  Subsystem1/1(vRef) -> [vRef]
  [speed] -> Sign1/1, Abs/1
  [Currents_dq_calc] -> ScopeIdIq/3
  [IqLim] -> SpeedController1/3(IqLim)
  Mean/1 -> Switch/3
  Saturation4/1 -> SpeedController/1(In1)
  Constant8/1 -> [Idreq]
  Min/1 -> Divide1/1
  Transfer Fcn5/1 -> Gain10/1, Scope/1
  Saturation3/1 -> Mean/1
  [P_dc] -> ScopeMain/7
  [speed] -> SpeedController/2(In2)
  Abs/1 -> 1-D Lookup Table3/1
  CurrentsMuxFilter1/1(Out1) -> Mux/1
  Mux8/1 -> ScopeDemag/2
  Subsystem1/5(Currents_work) -> [Currents_work]
  [Idreq] -> Mux6/2
  Constant5/1 -> Min/1
  [speed] -> Subsystem1/3(speed)
  Subsystem4/1(Voltages) -> [Voltages]
  Subsystem1/7(Ang) -> [AngleWork]
  [Iqreq] -> Mux6/1
  [Vdc] -> Transfer Fcn2/1
  Saturation1/1 -> Divide/2
  [angle_elec] -> Park Transform/2
  PS-Simulink Converter3/1 -> [Torque]
  Mux4/1 -> ScopeMain/3
  Transfer Fcn3/1 -> Abs1/1
  PS-Simulink Converter2/1 -> [speed]
  Gain10/1 -> SpeedController1/1(Idc_req)
  [Ud] -> Mux4/1
  Ramp2/1 -> Saturation4/1
  [IqReq1] -> Switch/1, Sum5/2
  Unit Delay2/1 -> [Kzi]
  [Voltages] -> CurrentsMuxFilter1/1(In1)
  Bias/1 -> Product3/1
  [IqLim] -> SpeedController/3(IqLim)
  [Currents] -> Clarke Transform/1
  Sign1/1 -> Product10/2
  Mux/1 -> ScopeMain/2
  Transfer Fcn4/1 -> Product2/2
  Sqrt1/1 -> Product1/2
  Switch/1 -> ScopeIqref/3, Saturation Dynamic/2
  Subsystem1/2(vAngle) -> [vAngle]
  Gain/1 -> Saturation Dynamic/3, ScopeIqref/2
  [Idreq] -> Square1/1
  [speed] -> Relational Operator/1
  [AngleWork] -> Park Transform1/2
  Sum5/1 -> Saturation3/1
  Abs3/1 -> Sqrt1/1
  Relational Operator/1 -> Data Type Conversion/1
  [Currents_dq_calc] -> Mux7/2
  Mean2/1 -> [P_dc]
  SpeedController1/1(IqReq) -> Scope/2, Product10/1
  Mux7/1 -> ScopeMain/4
  SVPWM1/4(vRefwork) -> Scope2/2
  [Uq] -> Transfer Fcn3/1
  SVPWM1/3(Tct) -> Mux5/3
  [vAngle] -> SVPWM1/2(vAngle)
  [Currents] -> CurrentsMuxFilter/1(In1)
  Gain3/1 -> [angle_elec]
  [vRef] -> Scope2/1, SVPWM1/1(vRef)
  [angle_elec] -> Subsystem1/2(angle)
  Transfer Fcn1/1 -> Square3/1
  Gain4/1 -> Saturation1/1
  [Torque] -> ScopeMain/6
  Subsystem4/2(Currents) -> [Currents]
  [Currents_work] -> Scope1/1, SVPWM1/4(Currents)
  Subsystem1/8(VDC) -> [VDCwork]
  Constant/1 -> Square/1
  [IqLim] -> Saturation Dynamic/1, ScopeIqref/1, Gain/1
  Park Transform1/1 -> ScopeIdIq/2
  Transfer Fcn2/1 -> Subsystem1/4(Vdc), Gain7/1
  Clock1/1 -> 1-D Lookup Table1/1
  Square1/1 -> Sum1/2
  Step/1 -> Bias/1, Switch/2
  Sum1/1 -> Saturation/1
  [speed] -> ScopeMain/5
  [Vdc] -> Divide1/2
  [Iqreq] -> Subsystem1/6(Iqreq)
  [Vdc] -> Product/2
  [Ud] -> Transfer Fcn1/1
  Sign/1 -> Product1/1
  [vRef] -> Mux4/3
  Subsystem1/3(Vd) -> [Ud]
  Gain8/1 -> Square2/1
  Square/1 -> Sum1/1
  Saturation/1 -> Sqrt/1
  Integrator/1 -> Scope7/1, Gain2/1
  Data Type Conversion/1 -> Transfer Fcn4/1
  Mux5/1 -> Scope1/2, Unit Delay2/1
  [IqLim] -> Mux8/1
  [I_dc] -> Product/1
  1-D Lookup Table1/1 -> ?
  connections:
  Capacitor/LConn1 -- Current Sensor13/RConn2 -- Voltage Sensor8/LConn1
  Ideal Semiconductor Switch1/LConn1 -- Half-Bridge Driver2/RConn1
  Half-Bridge Driver1/RConn1 -- Ideal Semiconductor Switch2/LConn1
  Current Sensor13/RConn1 -- PS-Simulink Converter9/LConn1
  Half-Bridge Driver2/RConn3 -- Ideal Semiconductor Switch3/LConn1
  Half-Bridge Driver/RConn1 -- Ideal Semiconductor Switch5/LConn1
  Voltage Sensor8/RConn1 -- PS-Simulink Converter10/LConn1
  Simulink-PS Converter5/RConn1 -- Half-Bridge Driver1/LConn1
  Ideal Semiconductor Switch6/LConn1 -- Half-Bridge Driver/RConn3
  Simulink-PS Converter/RConn1 -- Half-Bridge Driver2/LConn1
  Current Sensor14/RConn1 -- PS-Simulink Converter11/LConn1
  Half-Bridge Driver1/RConn3 -- Ideal Semiconductor Switch4/LConn1
  PS-Simulink Converter8/LConn1 -- Current Sensor2/RConn1
  Current Sensor2/LConn1 -- Current Sensor13/LConn1 -- Resistor3/LConn1
  DC Voltage Source/RConn1 -- Electrical Reference1/LConn1 -- Resistor1/RConn1
  Half-Bridge Driver1/RConn4 -- Ideal Semiconductor Switch4/RConn2 -- Half-Bridge Driver/RConn4 -- Ideal Semiconductor Switch6/RConn2 -- Solver Configuration1/RConn1 -- Voltage Sensor8/RConn2 -- Capacitor/RConn1 -- Resistor1/LConn1 -- Ideal Semiconductor Switch3/RConn2 -- Half-Bridge Driver2/RConn4
  Simulink-PS Converter7/RConn1 -- Half-Bridge Driver/LConn1
  Half-Bridge Driver1/RConn2 -- Connection Label3/LConn1 -- Ideal Semiconductor Switch4/RConn1 -- Ideal Semiconductor Switch2/RConn2
  Ideal Semiconductor Switch6/RConn1 -- Half-Bridge Driver/RConn2 -- Connection Label4/LConn1 -- Ideal Semiconductor Switch5/RConn2
  Half-Bridge Driver2/RConn2 -- Connection Label/LConn1 -- Ideal Semiconductor Switch3/RConn1 -- Ideal Semiconductor Switch1/RConn2
  Ideal Semiconductor Switch1/RConn1 -- Ideal Semiconductor Switch5/RConn1 -- Ideal Semiconductor Switch2/RConn1 -- Current Sensor2/RConn2
  Resistor3/RConn1 -- Inductor/RConn1
  Resistor2/RConn1 -- Current Sensor14/LConn1
  Current Sensor14/RConn2 -- Inductor/LConn1
  DC Voltage Source/LConn1 -- Resistor2/LConn1
  Ideal Torque Source/RConn2 -- Mechanical Rotational Reference3/LConn1 -- Ideal Torque Source/LConn1 -- Ideal Angular Velocity Source/RConn2
  Ideal Rotational Motion Sensor/LConn1 -- Ideal Torque Sensor/LConn1 -- PMSM/RConn1
  Inertia/LConn1 -- Ideal Torque Sensor/RConn1 -- Ideal Angular Velocity Source/LConn1
  Simulink-PS Converter2/RConn1 -- Ideal Torque Source/RConn1
  PMSM/LConn2 -- Subsystem4/RConn2
  Connection Label9/LConn1 -- Subsystem4/LConn1
  PS-Simulink Converter3/LConn1 -- Ideal Torque Sensor/RConn2
  PMSM/LConn3 -- Subsystem4/RConn3
  PS-Simulink Converter1/LConn1 -- Ideal Rotational Motion Sensor/RConn3
  Ideal Rotational Motion Sensor/RConn1 -- Mechanical Rotational Reference2/LConn1
  PMSM/RConn2 -- Mechanical Rotational Reference/LConn1
  PMSM/LConn1 -- Subsystem4/RConn1
  Connection Label1/LConn1 -- Subsystem4/LConn3
  PS-Simulink Converter2/LConn1 -- Ideal Rotational Motion Sensor/RConn2
  Simulink-PS Converter1/RConn1 -- Ideal Angular Velocity Source/RConn1
  Connection Label2/LConn1 -- Subsystem4/LConn2

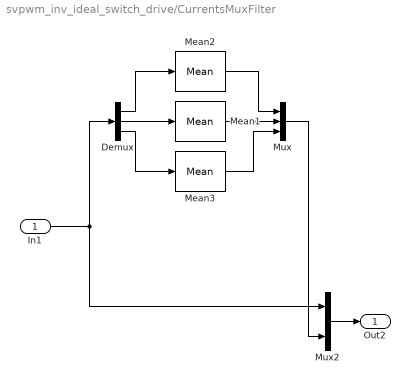
== system svpwm_inv_ideal_switch_drive/CurrentsMuxFilter ==
  In1 : Inport
  Demux : Demux  Outputs=3
  Mean1 : spsMeanLib/Mean  Freq=20000  Vinit=0  Ts=0
  Mean2 : spsMeanLib/Mean  Freq=20000  Vinit=0  Ts=0
  Mean3 : spsMeanLib/Mean  Freq=20000  Vinit=0  Ts=0
  Mux : Mux  Inputs=3
  Mux2 : Mux  Inputs=2
  Out2 : Outport
  wires:
  Mean3/1 -> Mux/3
  Mean1/1 -> Mux/2
  Mean2/1 -> Mux/1
  Demux/3 -> Mean3/1
  Demux/2 -> Mean1/1
  Demux/1 -> Mean2/1
  Mux2/1 -> Out2/1
  In1/1 -> Mux2/1, Demux/1
  Mux/1 -> Mux2/2

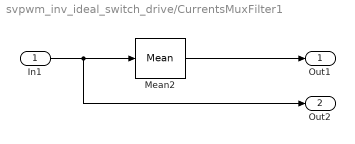
== system svpwm_inv_ideal_switch_drive/CurrentsMuxFilter1 ==
  In1 : Inport
  Mean2 : spsMeanLib/Mean  Freq=20000  Vinit=0  Ts=0
  Out1 : Outport
  Out2 : Outport  Port=2
  wires:
  In1/1 -> Mean2/1, Out2/1
  Mean2/1 -> Out1/1

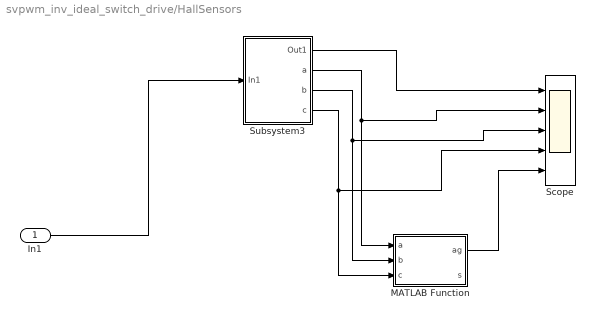
== system svpwm_inv_ideal_switch_drive/HallSensors ==
  In1 : Inport
  MATLAB Function : MATLAB Function  TreatAsAtomicUnit=on  SystemSampleTime=1/40000
  Scope : Scope  NumInputPorts=5
      settings: ActiveDisplayYMinimum=-0.7854  ActiveDisplayYMaximum=7.06858  DataLoggingVariableName=ScopeData3
  Subsystem3 : Subsystem
  wires:
  In1/1 -> Subsystem3/1(In1)
  Subsystem3/3(b) -> MATLAB Function/2(b), Scope/3
  MATLAB Function/1(ag) -> Scope/5
  Subsystem3/2("a ") -> MATLAB Function/1(a), Scope/2
  Subsystem3/4(c) -> MATLAB Function/3(c), Scope/4
  Subsystem3/1(Out1) -> Scope/1

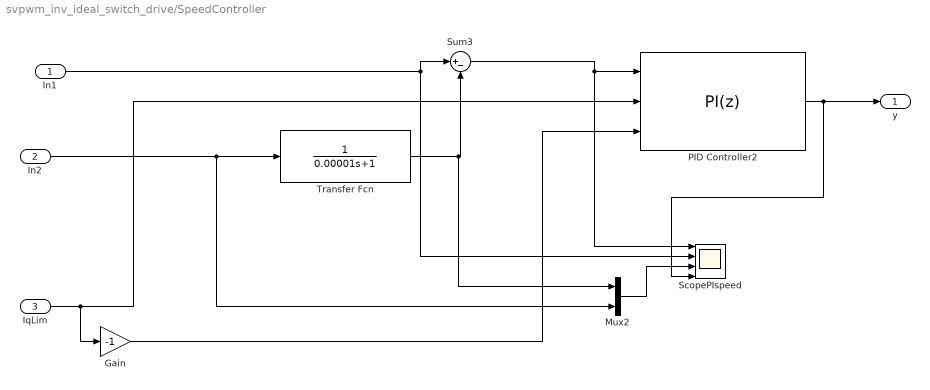
== system svpwm_inv_ideal_switch_drive/SpeedController ==
  In1 : Inport
  In2 : Inport  Port=2
  IqLim : Inport  Port=3
  Gain : Gain  Gain=-1
  Mux2 : Mux  Inputs=2
  PID Controller2 : slpidlib/PID Controller  Controller=PI  Form=Parallel  TimeDomain=Discrete-time  UseExternalTs=off  SampleTime=FocDiscrTime  IntegratorMethod=Forward Euler  FilterMethod=Forward Euler  ControllerParametersSource=internal  P=5  I=1  UseKiTs=off  D=0  UseExternalDerivativeSource=off  N=100  UseFilter=on  TunerSelectOption=Transfer Function Based (PID Tuner App)  InitialConditionSource=internal  InitialConditionForIntegrator=0  InitialConditionForFilter=0  DifferentiatorICPrevScaledInput=0  ExternalReset=none  TrackingMode=off  Kt=1  LimitOutput=on  SatLimitsSource=external  UpperSaturationLimit=350  LowerSaturationLimit=-3  LinearizeAsGain=on  AntiWindupMode=clamping  Kb=1  LimitIntegrator=off  UpperIntegratorSaturationLimit=inf  LowerIntegratorSaturationLimit=-inf  POutMin=[]  POutMax=[]  IOutMin=[]  IOutMax=[]  DOutMin=[]  DOutMax=[]  NOutMin=[]  NOutMax=[]  SumOutMin=[]  SumOutMax=[]  SaturationOutMin=[]  SaturationOutMax=[]  PParamMin=[]  PParamMax=[]  IParamMin=[]  IParamMax=[]  DParamMin=[]  DParamMax=[]  NParamMin=[]  NParamMax=[]  KbParamMin=[]  KbParamMax=[]  KtParamMin=[]  KtParamMax=[]  KbOutMin=[]  KbOutMax=[]  KtOutMin=[]  KtOutMax=[]  IntegratorOutMin=[]  IntegratorOutMax=[]  FilterOutMin=[]  FilterOutMax=[]  SumI1OutMin=[]  SumI1OutMax=[]  SumI2OutMin=[]  SumI2OutMax=[]  SumI3OutMin=[]  SumI3OutMax=[]  SumI4OutMin=[]  SumI4OutMax=[]  SumDOutMin=[]  SumDOutMax=[]  DifferentiatorOutMin=[]  DifferentiatorOutMax=[]  FilterDiffOutCoefMin=[]  FilterDiffOutCoefMax=[]  ReciprocalOutMin=[]  ReciprocalOutMax=[]  SumDenOutMin=[]  SumDenOutMax=[]  SumNumOutMin=[]  SumNumOutMax=[]  DivideOutMin=[]  DivideOutMax=[]  UdiffTsProdOutMin=[]  UdiffTsProdOutMax=[]  NTsProdOutMin=[]  NTsProdOutMax=[]  UintegralTsProdOutMin=[]  UintegralTsProdOutMax=[]  UngainTsProdOutMin=[]  UngainTsProdOutMax=[]  ClampingZeroOutDataTypeStr=Inherit: Inherit via back propagation  ClampingZeroOutMin=[]  ClampingZeroOutMax=[]  FilterDenConstantOutDataTypeStr=Inherit: Inherit via back propagation  FilterDenConstantOutMin=[]  FilterDenConstantOutMax=[]  PCopyOutDataTypeStr=Inherit: Inherit via back propagation  PCopyOutMin=[]  PCopyOutMax=[]  NCopyOutDataTypeStr=Inherit: Inherit via back propagation  NCopyOutMin=[]  NCopyOutMax=[]  IntegratorContinuousStateAttributes=''  IntegratorStateMustResolveToSignalObject=off  IntegratorRTWStateStorageClass=Auto  FilterContinuousStateAttributes=''  FilterStateMustResolveToSignalObject=off  FilterRTWStateStorageClass=Auto  ParallelPVariant=InternalParameters  IdealPVariant=Disabled  IVariant=InternalParameters  DVariant=Disabled  IntegratorVariant=Discrete  SatVariant=External  AWVariant=DiscClampingParallel  PCopyVariant=Disabled  TRVariant=Disabled  FdbkBlocksVariant=Forward  IdealPFdbkVariant=Disabled  SatFdbkVariant=Disabled  DerivativeFilterVariant=Disabled  NVariant=Disabled  NCopyVariant=Disabled_SignalSpec  FilterICVariant=Disabled  IntegratorICVariant=InternalICs  ExternalResetVariant=Disabled  TRSumVariant=Passthrough  SumFdbkVariant=Disabled  SumVariant=Sum_PI  TsampFilterVariant=InternalTs  TsampNgainVariant=Passthrough  TsampIntegralVariant=Disabled_SignalSpec  ExternalSaturationOutDataTypeStr=Inherit: Same as second input  DerivativeSourceVariant=Disabled  PreIntVariant=InternalPreInt
  ScopePIspeed : Scope  NumInputPorts=4
      settings: ActiveDisplayYMinimum=-74.846087618837728  ActiveDisplayYMaximum=672.6746403902182  DataLoggingVariableName=ScopeData10
  Sum3 : Sum  Inputs=|+-
  Transfer Fcn : TransferFcn  Denominator=[0.00001 1]
  y : Outport
  wires:
  Mux2/1 -> ScopePIspeed/3
  In2/1 -> Mux2/2, Transfer Fcn/1
  PID Controller2/1 -> y/1, ScopePIspeed/4
  Sum3/1 -> ScopePIspeed/1, PID Controller2/1
  Transfer Fcn/1 -> Mux2/1, Sum3/2
  In1/1 -> Sum3/1, ScopePIspeed/2
  IqLim/1 -> Gain/1, PID Controller2/2
  Gain/1 -> PID Controller2/3

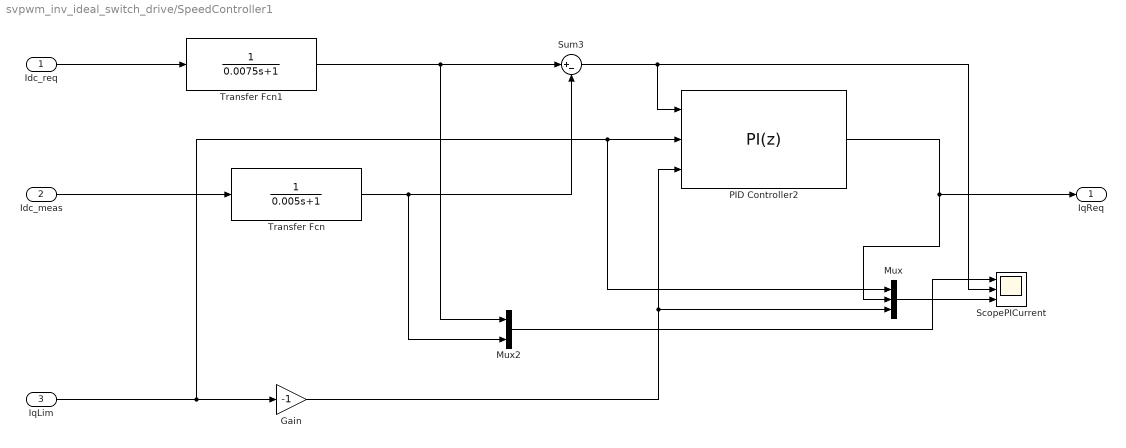
== system svpwm_inv_ideal_switch_drive/SpeedController1 ==
  Idc_req : Inport
  Idc_meas : Inport  Port=2
  IqLim : Inport  Port=3
  Gain : Gain  Gain=-1
  Mux : Mux  Inputs=3
  Mux2 : Mux  Inputs=2
  PID Controller2 : slpidlib/PID Controller  Controller=PI  Form=Parallel  TimeDomain=Discrete-time  UseExternalTs=off  SampleTime=FocDiscrTime  IntegratorMethod=Forward Euler  FilterMethod=Forward Euler  ControllerParametersSource=internal  P=5  I=450  UseKiTs=off  D=0  UseExternalDerivativeSource=off  N=100  UseFilter=on  TunerSelectOption=Transfer Function Based (PID Tuner App)  InitialConditionSource=internal  InitialConditionForIntegrator=0  InitialConditionForFilter=0  DifferentiatorICPrevScaledInput=0  ExternalReset=none  TrackingMode=off  Kt=1  LimitOutput=on  SatLimitsSource=external  UpperSaturationLimit=350  LowerSaturationLimit=-3  LinearizeAsGain=on  AntiWindupMode=clamping  Kb=1  LimitIntegrator=off  UpperIntegratorSaturationLimit=inf  LowerIntegratorSaturationLimit=-inf  POutMin=[]  POutMax=[]  IOutMin=[]  IOutMax=[]  DOutMin=[]  DOutMax=[]  NOutMin=[]  NOutMax=[]  SumOutMin=[]  SumOutMax=[]  SaturationOutMin=[]  SaturationOutMax=[]  PParamMin=[]  PParamMax=[]  IParamMin=[]  IParamMax=[]  DParamMin=[]  DParamMax=[]  NParamMin=[]  NParamMax=[]  KbParamMin=[]  KbParamMax=[]  KtParamMin=[]  KtParamMax=[]  KbOutMin=[]  KbOutMax=[]  KtOutMin=[]  KtOutMax=[]  IntegratorOutMin=[]  IntegratorOutMax=[]  FilterOutMin=[]  FilterOutMax=[]  SumI1OutMin=[]  SumI1OutMax=[]  SumI2OutMin=[]  SumI2OutMax=[]  SumI3OutMin=[]  SumI3OutMax=[]  SumI4OutMin=[]  SumI4OutMax=[]  SumDOutMin=[]  SumDOutMax=[]  DifferentiatorOutMin=[]  DifferentiatorOutMax=[]  FilterDiffOutCoefMin=[]  FilterDiffOutCoefMax=[]  ReciprocalOutMin=[]  ReciprocalOutMax=[]  SumDenOutMin=[]  SumDenOutMax=[]  SumNumOutMin=[]  SumNumOutMax=[]  DivideOutMin=[]  DivideOutMax=[]  UdiffTsProdOutMin=[]  UdiffTsProdOutMax=[]  NTsProdOutMin=[]  NTsProdOutMax=[]  UintegralTsProdOutMin=[]  UintegralTsProdOutMax=[]  UngainTsProdOutMin=[]  UngainTsProdOutMax=[]  ClampingZeroOutDataTypeStr=Inherit: Inherit via back propagation  ClampingZeroOutMin=[]  ClampingZeroOutMax=[]  FilterDenConstantOutDataTypeStr=Inherit: Inherit via back propagation  FilterDenConstantOutMin=[]  FilterDenConstantOutMax=[]  PCopyOutDataTypeStr=Inherit: Inherit via back propagation  PCopyOutMin=[]  PCopyOutMax=[]  NCopyOutDataTypeStr=Inherit: Inherit via back propagation  NCopyOutMin=[]  NCopyOutMax=[]  IntegratorContinuousStateAttributes=''  IntegratorStateMustResolveToSignalObject=off  IntegratorRTWStateStorageClass=Auto  FilterContinuousStateAttributes=''  FilterStateMustResolveToSignalObject=off  FilterRTWStateStorageClass=Auto  ParallelPVariant=InternalParameters  IdealPVariant=Disabled  IVariant=InternalParameters  DVariant=Disabled  IntegratorVariant=Discrete  SatVariant=External  AWVariant=DiscClampingParallel  PCopyVariant=Disabled  TRVariant=Disabled  FdbkBlocksVariant=Forward  IdealPFdbkVariant=Disabled  SatFdbkVariant=Disabled  DerivativeFilterVariant=Disabled  NVariant=Disabled  NCopyVariant=Disabled_SignalSpec  FilterICVariant=Disabled  IntegratorICVariant=InternalICs  ExternalResetVariant=Disabled  TRSumVariant=Passthrough  SumFdbkVariant=Disabled  SumVariant=Sum_PI  TsampFilterVariant=InternalTs  TsampNgainVariant=Passthrough  TsampIntegralVariant=Disabled_SignalSpec  ExternalSaturationOutDataTypeStr=Inherit: Same as second input  DerivativeSourceVariant=Disabled  PreIntVariant=InternalPreInt
  ScopePICurrent : Scope  NumInputPorts=3
      settings: ActiveDisplayYMinimum=-115.94774316156257  ActiveDisplayYMaximum=12.883155082671625  DataLoggingVariableName=ScopeData10
  Sum3 : Sum  Inputs=|+-
  Transfer Fcn : TransferFcn  Denominator=[0.005 1]
  Transfer Fcn1 : TransferFcn  Denominator=[0.0075 1]
  IqReq : Outport
  wires:
  Idc_req/1 -> Transfer Fcn1/1
  Transfer Fcn/1 -> Sum3/2, Mux2/2
  Sum3/1 -> PID Controller2/1, ScopePICurrent/2
  Mux2/1 -> ScopePICurrent/1
  Idc_meas/1 -> Transfer Fcn/1
  PID Controller2/1 -> Mux/2, IqReq/1
  IqLim/1 -> PID Controller2/2, Mux/1, Gain/1
  Gain/1 -> PID Controller2/3, Mux/3
  Transfer Fcn1/1 -> Mux2/1, Sum3/1
  Mux/1 -> ScopePICurrent/3
